simulink model "Integrated_Project"  (R2025b)
settings: Solver=ode1  StartTime=0.0  StopTime=1400  FixedStep=0.1  RelTol=1e-3
model workspace (MAT data in the model file):
  front_gain_calibration = 0.772532167539
  left_gain_calibration = 5
  right_gain_calibration = 6
values from neighbouring files (symbols this model uses):
  a_current = exp(-Ts/tau_current)    [Integrated_Project_Script.m]
  a_turn = exp(-0.1/0.5)    [Integrated_Project_Script.m]
  Charging_Current = -25    [Integrated_Project_Script.m]
  omega_TURN = double(0.5)    [Integrated_Project_Script.m]
  SOC_Critical = double(5)    [Integrated_Project_Script.m]
  SOC_Warn = double(30)    [Integrated_Project_Script.m]
  SOH_Min = double(90)    [Integrated_Project_Script.m]
  V_min = double(2.5)    [Integrated_Project_Script.m]
  vx_FORWARD = double(0.5)    [Integrated_Project_Script.m]
  vx_REDUCED = double(0.2)    [Integrated_Project_Script.m]
undefined symbols (not defined in the file or in its folder): DiscIntNeverNeededParam, dspblkCoreblockFVToolHelper, gcbh
libraries: simulink x6, sim3dlib x1, sim3dautolib x1, SignalEditorBlockLib x1
settings Model: VariantFading=off  Creator=LENOVO  LastModifiedBy=LENOVO

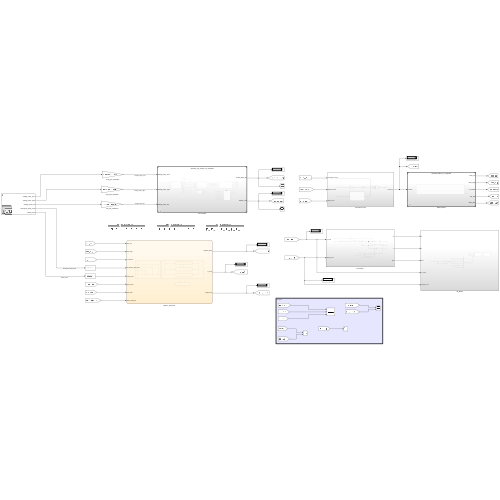
[thumbnail: Simulink's stored preview of the top-level diagram]
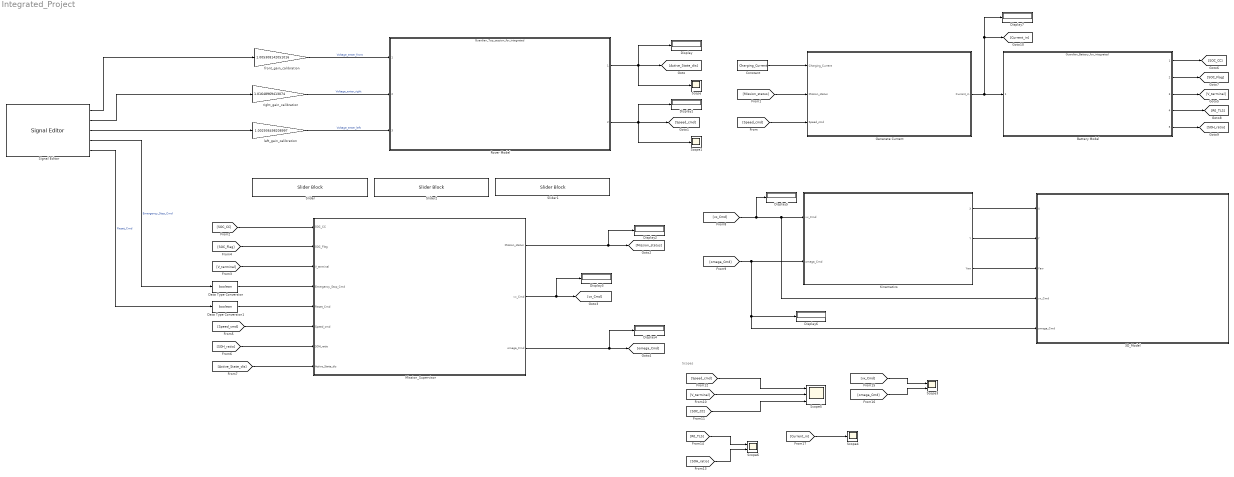
== system Integrated_Project ==
  note: Scopes
  3D_Model : Subsystem
  Battery Model : ModelReference  ModelNameDialog=Guardian_Battery_for_integrated.slx  SimulationMode=Normal  ModelReferenceVersion=1.37
  Constant : Constant  Value=Charging_Current
  Data Type Conversion : DataTypeConversion  OutDataTypeStr=boolean  SaturateOnIntegerOverflow=off  RndMeth=Floor
  Data Type Conversion1 : DataTypeConversion  OutDataTypeStr=boolean  SaturateOnIntegerOverflow=off  RndMeth=Floor
  Display{,1..7} (8 alike) : Display
  Generate Current : Subsystem
  Kinematics : Subsystem
  Mission_Supervisor : Stateflow chart  TreatAsAtomicUnit=on
  Rover Model : ModelReference  ModelNameDialog=Guardian_Top_session_for_integrated.slx  SimulationMode=Normal  ModelReferenceVersion=1.68
  Scope : Scope
  Scope1 : Scope
  Scope3 : Scope  NumInputPorts=2
      settings: ActiveDisplayYMinimum=-0.625  ActiveDisplayYMaximum=0.625  DataLoggingVariableName=ScopeData3
  Scope4 : Scope
      settings: ActiveDisplayYMinimum=-33.124999999999993  ActiveDisplayYMaximum=48.124999999999936  DataLoggingVariableName=ScopeData4
  Scope5 : Scope  NumInputPorts=3
      settings: ActiveDisplayString=3  ActiveDisplayYMinimum=45.574520890625735  ActiveDisplayYMaximum=83.82505323437492  DataLoggingVariableName=ScopeData6
  Scope6 : Scope  NumInputPorts=2
      settings: ActiveDisplayYMinimum=-1  ActiveDisplayYMaximum=1  DataLoggingVariableName=ScopeData7
  Signal Editor : SignalEditorBlockLib/Signal Editor  FileName=scenario_FINAL_ceremony.mat  ActiveScenario=ds  ActiveSignal=Voltage_enter_front  IsBus=off  OutputBusObjectStr=Bus: BusObject  SampleTime=0  ZeroCross=off  OutputAfterFinalValue=Setting to zero  Unit=inherit  PreserveSignalName=on  ApplySigPropsToAllScenarios=on  ApplySigPropsToAllSignals=off  SignalPropertySource=Dialog parameters
  Slider : SliderBlock  ScaleMax=3
  Slider1 : SliderBlock  ScaleMax=3
  Slider2 : SliderBlock  ScaleMax=3
  front_gain_calibration : Gain  Gain=1.005308142051016
  left_gain_calibration : Gain  Gain=1.002936498208997
  right_gain_calibration : Gain  Gain=1.01648969413074
  wires:
  left_gain_calibration/1 -> Rover Model/3  "Voltage_enter_left"
  front_gain_calibration/1 -> Rover Model/1  "Voltage_enter_front"
  right_gain_calibration/1 -> Rover Model/2  "Voltage_enter_right"
  Signal Editor/1 -> front_gain_calibration/1
  Signal Editor/2 -> right_gain_calibration/1
  Signal Editor/3 -> left_gain_calibration/1
  Rover Model/1 -> Display/1, Scope/1, [Active_State_dis]
  Rover Model/2 -> Scope1/1, Display1/1, [Speed_cmd]
  Signal Editor/5 -> Data Type Conversion1/1  "Reset_Cmd"
  Signal Editor/4 -> Data Type Conversion/1  "Emergency_Stop_Cmd"
  Data Type Conversion/1 -> Mission_Supervisor/4(Emergency_Stop_Cmd)
  Data Type Conversion1/1 -> Mission_Supervisor/5(Reset_Cmd)
  Mission_Supervisor/1(Mission_status) -> Display2/1, [Mission_status]
  Mission_Supervisor/2(vx_Cmd) -> Display3/1, [vx_Cmd]
  Mission_Supervisor/3(omega_Cmd) -> Display4/1, [omega_Cmd]
  [Mission_status] -> Generate Current/2(Mission_status)
  [Speed_cmd] -> Generate Current/3(Speed_cmd)
  Constant/1 -> Generate Current/1(Charging_Current)
  Generate Current/1(Current_in) -> [Current_in], Display7/1, Battery Model/1
  Battery Model/1 -> [SOC_CC]
  Battery Model/2 -> [SOC_Flag]
  Battery Model/3 -> [V_terminal]
  Battery Model/4 -> [R0_TLS]
  Battery Model/5 -> [SOH_ratio]
  [SOC_CC] -> Mission_Supervisor/1(SOC_CC)
  [V_terminal] -> Mission_Supervisor/3(V_terminal)
  [SOC_Flag] -> Mission_Supervisor/2(SOC_Flag)
  [Speed_cmd] -> Mission_Supervisor/6(Speed_cmd)
  [SOH_ratio] -> Mission_Supervisor/7(SOH_ratio)
  [Active_State_dis] -> Mission_Supervisor/8(Active_State_dis)
  [vx_Cmd] -> Display5/1, 3D_Model/4(vx_Cmd), Kinematics/1(vx_Cmd)
  [omega_Cmd] -> Display6/1, 3D_Model/5(omega_Cmd), Kinematics/2(omega_Cmd)
  Kinematics/1(X) -> 3D_Model/1(X)
  Kinematics/2(Y) -> 3D_Model/2(Y)
  Kinematics/3(Yaw) -> 3D_Model/3(Yaw)
  [Speed_cmd] -> Scope5/1
  [V_terminal] -> Scope5/2
  [SOC_CC] -> Scope5/3
  [R0_TLS] -> Scope6/1
  [SOH_ratio] -> Scope6/2
  [vx_Cmd] -> Scope3/1
  [omega_Cmd] -> Scope3/2
  [Current_in] -> Scope4/1

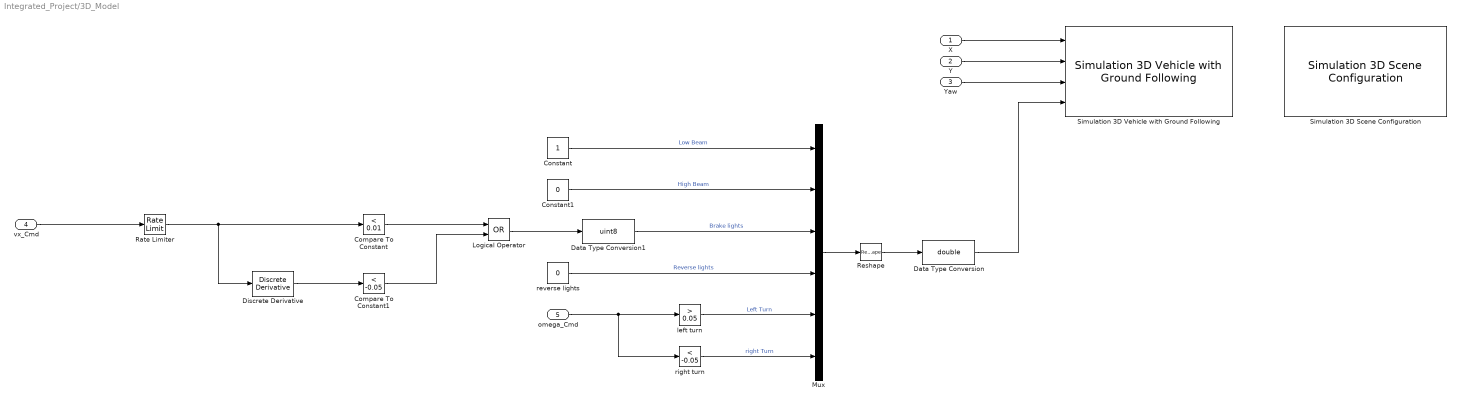
== system Integrated_Project/3D_Model ==
  X : Inport
  Y : Inport  Port=2
  Yaw : Inport  Port=3
  vx_Cmd : Inport  Port=4
  omega_Cmd : Inport  Port=5
  Compare To Constant : simulink/Logic and Bit Operations/Compare To Constant  relop=<  const=0.01  OutDataTypeStr=uint8
  Compare To Constant1 : simulink/Logic and Bit Operations/Compare To Constant  relop=<  const=-0.05  OutDataTypeStr=boolean
  Constant : Constant  OutDataTypeStr=uint8
  Constant1 : Constant  Value=0  OutDataTypeStr=uint8
  Data Type Conversion : DataTypeConversion  OutDataTypeStr=double  SaturateOnIntegerOverflow=off  RndMeth=Floor
  Data Type Conversion1 : DataTypeConversion  OutDataTypeStr=uint8  SaturateOnIntegerOverflow=off  RndMeth=Floor
  Discrete Derivative : simulink/Discrete/Discrete Derivative  gainval=1.0  ICPrevScaledInput=0.0  OutMin=[]  OutMax=[]  OutDataType=fixdt(1, 16)  OutScaling=2^-10  DoSatur=off
  Logical Operator : Logic  Operator=OR  AllPortsSameDT=off  OutDataTypeStr=boolean
  Mux : Mux  Inputs=6
  Rate Limiter : RateLimiter  RisingSlewLimit=0.5  SampleTimeMode=inherited
  Reshape : Reshape  OutputDimensions=[1 , 6]
  Simulation 3D Scene Configuration : sim3dlib/Simulation 3D Scene Configuration  Priority=0  ProjectFormat=Default Scenes  SceneDesc=Straight road  ProjectName=C:\Program Files\MATLAB\R2025b\toolbox\shared\sim3d_projects\automotive_project_windows\UE\WindowsNoEditor\VehicleSimulation.exe  ScenePath=/Game/Maps/HwStrght  EnableOpenDRIVE=off  vehTagList={'Custom';'NAGY';'Scene Origin'}  vehTag=NAGY  AttachedCameraRelativeTranslation=[0 0 0]  FreeCameraDefaultInitialTranslation=[-6, 0, 2]  AttachedCameraRelativeRotation=[0 0 0]  FreeCameraDefaultInitialRotation=[0, -15, 0]  ViewpointName=Custom  FreeCameraInitialTranslation=[0, 0, 0]  ViewpointTranslation=[0 0 0]  FreeCameraInitialRotation=[0, 0, 0]  ViewpointRotation=[0 0 0]  OpVisEn=off  Ts=0.1  EnableWindow=on  EnableRemoteAccess=off  EnableWeather=on  SunAzimuth=0.0  SunAltitude=18.0  EnableGeospatialSun=off  Latitude=0  Longitude=0  Date=2023-01-01  Time=10:30:00  GeoTimeZone=-5.0  SunDaylightSaving=off  wind=1  clouds=10  EnableVolumetricClouds=off  CloudCoverage=0  CloudAltitude=6  fog=0  rain=0  RaindropsEffect=off  SnowDensity=0  EnableGeospatial=off  TilesetSource=Earth terrain  UseTrueOrigin=off  OriginHeight=200  OriginLatitude=40.744652  OriginLongitude=-73.988864  MapStyle=Aerial  AdditionalAssetIDs=[]  UseAdvancedSunSky=off  SolarTime=11  TimeZone=-5  Day=21  Month=9  Year=2022  UseDaylightSavingTime=on  DSTStartDay=10  DSTStartMonth=3  DSTEndDay=3  DSTEndMonth=11  DSTSwitchHour=2  sensorTag=MainCamera1  sensorId=1  sensorName=MainCamera1  mountLoc=Origin  offsetFlag=off  tmountOffset=[0, 0, 0]  rmountOffset=[0, 0, 0]  HorizontalResolution=1280  VerticalResolution=720  HorizontalFOV=60  mountPoint=[0 0 0]  mountOrientation=[0 0 0]  aMode=5  ID=1  GeoTrigger=Inactive  ViewNameList={'Custom'}  ViewTranslationList={'[0 0 0]'}  ViewRotationList={'[0 0 0]'}
      settings: LibrarySourceBlock=sl3dlib/Simulation 3D/Environment/Simulation 3D Scene Configuration
  Simulation 3D Vehicle with Ground Following : sim3dautolib/Simulation 3D Vehicle with Ground Following  Priority=-1  PassVehMesh=Muscle car  MeshPath=/MathWorksAutomotiveContent/Vehicles/Muscle/Meshes/SK_MuscleCar.SK_MuscleCar  TrackWidth=1.9  WheelBase=3  WheelRadius=0.35  VehColor=Black  CoordinateSystem=ISO8855  InitialPos=[0, 0, 0]  InitialRot=[0, 0, 0]  ActorName=NAGY  SampleTime=0.1  ActorType=SimulinkVehicle  ID=C  aMode=3  ActorTag=NAGY  CoordinateScheme=0  VehLightsControl=on  HeadlightColor=[ 1, 0.95 , 0.7 ]  HighBeamIntensity=60000  LowBeamIntensity=20000  HighBeamConeAngle=35  LowBeamConeAngle=35  LeftHeadlightOrientation=[ -5, 0 ]  RightHeadlightOrientation=[ -5, 0 ]  BrakelightIntensity=1500  ReverselightIntensity=1500  SignallightIntensity=5000  SignallightPeriod=0.8  SignalPulseWidth=50  TransformOutportEnabled=off
      settings: LibrarySourceBlock=drivingsim3d/Simulation 3D Vehicle with Ground Following
  left turn : simulink/Logic and Bit Operations/Compare To Constant  relop=>  const=0.05  OutDataTypeStr=uint8
  reverse lights : Constant  Value=0  OutDataTypeStr=uint8
  right turn : simulink/Logic and Bit Operations/Compare To Constant  relop=<  const=-0.05  OutDataTypeStr=uint8
  wires:
  Yaw/1 -> Simulation 3D Vehicle with Ground Following/3
  Y/1 -> Simulation 3D Vehicle with Ground Following/2
  X/1 -> Simulation 3D Vehicle with Ground Following/1
  Data Type Conversion/1 -> Simulation 3D Vehicle with Ground Following/4
  Constant1/1 -> Mux/2  "High Beam"
  right turn/1 -> Mux/6  "right Turn"
  reverse lights/1 -> Mux/4  "Reverse lights"
  omega_Cmd/1 -> right turn/1, left turn/1
  Constant/1 -> Mux/1  "Low Beam"
  Compare To Constant/1 -> Logical Operator/1
  Mux/1 -> Reshape/1
  vx_Cmd/1 -> Rate Limiter/1
  left turn/1 -> Mux/5  "Left Turn"
  Reshape/1 -> Data Type Conversion/1
  Rate Limiter/1 -> Discrete Derivative/1, Compare To Constant/1
  Logical Operator/1 -> Data Type Conversion1/1
  Discrete Derivative/1 -> Compare To Constant1/1
  Compare To Constant1/1 -> Logical Operator/2
  Data Type Conversion1/1 -> Mux/3  "Brake lights"

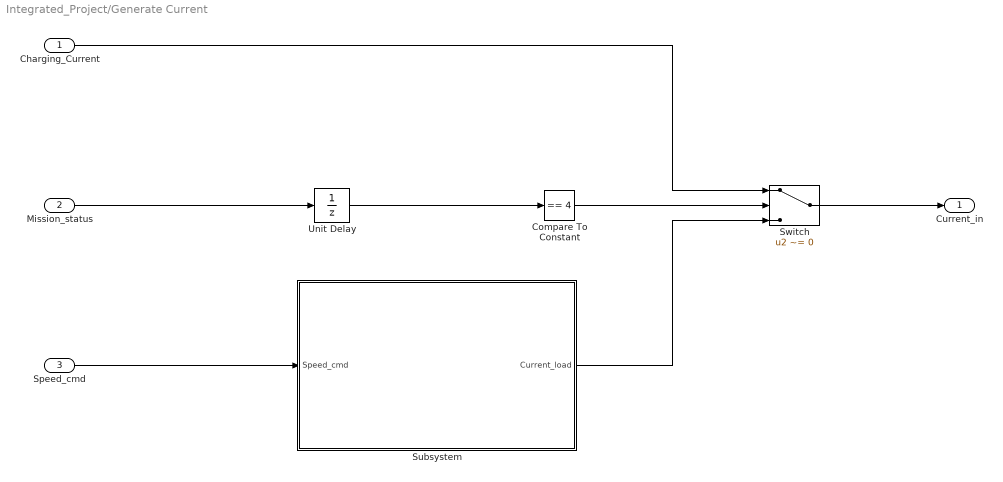
== system Integrated_Project/Generate Current ==
  Charging_Current : Inport
  Mission_status : Inport  Port=2
  Speed_cmd : Inport  Port=3
  Compare To Constant : simulink/Logic and Bit Operations/Compare To Constant  relop===  const=4  OutDataTypeStr=boolean
  Subsystem : Subsystem
  Switch : Switch  Criteria=u2 ~= 0  Threshold=4  SaturateOnIntegerOverflow=off  InputSameDT=off
  Unit Delay : UnitDelay  SampleTime=-1  HasFrameUpgradeWarning=on
  Current_in : Outport
  wires:
  Mission_status/1 -> Unit Delay/1
  Unit Delay/1 -> Compare To Constant/1
  Compare To Constant/1 -> Switch/2
  Charging_Current/1 -> Switch/1
  Speed_cmd/1 -> Subsystem/1(Speed_cmd)
  Subsystem/1(Current_load) -> Switch/3
  Switch/1 -> Current_in/1

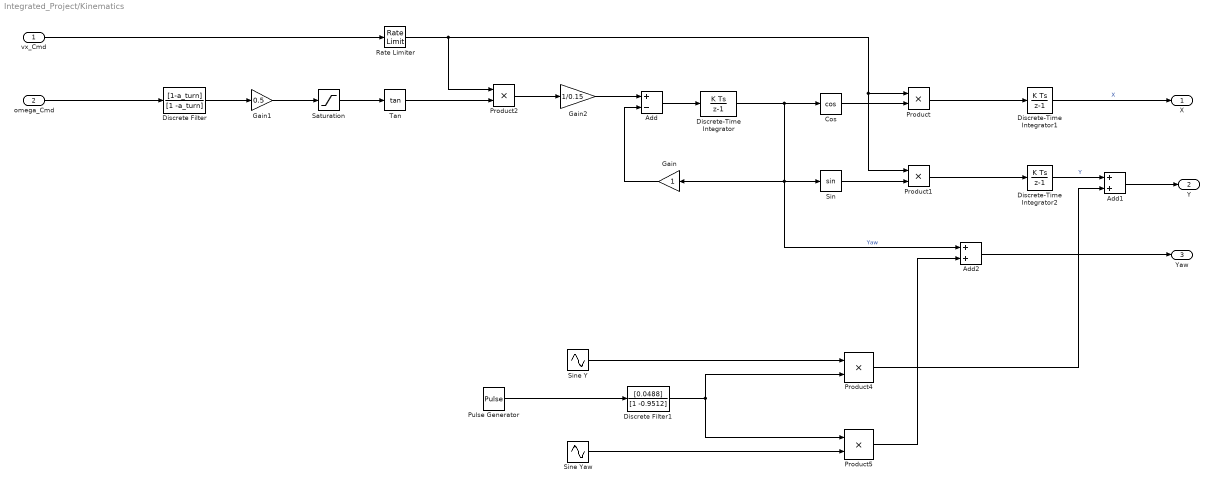
== system Integrated_Project/Kinematics ==
  vx_Cmd : Inport
  omega_Cmd : Inport  Port=2
  Add : Sum  Inputs=+-
  Add1 : Sum
  Add2 : Sum
  Cos : Trigonometry  Operator=cos
  Discrete Filter : DiscreteFilter  LoadFcn=dspblkCoreblockFVToolHelper(gcbh,'load');  Numerator=[1-a_turn]  Denominator=[1 -a_turn]
      settings: CopyFcn=dspblkCoreblockFVToolHelper(gcbh,'copy');  DeleteFcn=dspblkCoreblockFVToolHelper(gcbh,'close');  ModelCloseFcn=dspblkCoreblockFVToolHelper(gcbh,'close');  PreSaveFcn=dspblkCoreblockFVToolHelper(gcbh,'presave');  PostSaveFcn=dspblkCoreblockFVToolHelper(gcbh,'postsave');  CloseFcn=dspblkCoreblockFVToolHelper(gcbh,'close');
  Discrete Filter1 : DiscreteFilter  LoadFcn=dspblkCoreblockFVToolHelper(gcbh,'load');  Numerator=[0.0488]  Denominator=[1 -0.9512]
      settings: CopyFcn=dspblkCoreblockFVToolHelper(gcbh,'copy');  DeleteFcn=dspblkCoreblockFVToolHelper(gcbh,'close');  ModelCloseFcn=dspblkCoreblockFVToolHelper(gcbh,'close');  PreSaveFcn=dspblkCoreblockFVToolHelper(gcbh,'presave');  PostSaveFcn=dspblkCoreblockFVToolHelper(gcbh,'postsave');  CloseFcn=dspblkCoreblockFVToolHelper(gcbh,'close');
  Discrete-Time Integrator : DiscreteIntegrator  SampleTime=-1  LimitOutput=on  UpperSaturationLimit=0.4  LowerSaturationLimit=-0.4  ICPrevOutput=DiscIntNeverNeededParam  ICPrevScaledInput=DiscIntNeverNeededParam
  Discrete-Time Integrator1 : DiscreteIntegrator  SampleTime=-1  ICPrevOutput=DiscIntNeverNeededParam  ICPrevScaledInput=DiscIntNeverNeededParam
  Discrete-Time Integrator2 : DiscreteIntegrator  SampleTime=-1  ICPrevOutput=DiscIntNeverNeededParam  ICPrevScaledInput=DiscIntNeverNeededParam
  Gain : Gain
  Gain1 : Gain  Gain=0.5
  Gain2 : Gain  Gain=1/0.15
  Product{,1..2,4..5} (5 alike) : Product
  Pulse Generator : DiscretePulseGenerator  PulseType=Time based  Period=1000  PulseWidth=2.4  PhaseDelay=30
  Rate Limiter : RateLimiter  RisingSlewLimit=0.5  SampleTimeMode=inherited
  Saturation : Saturate
  Sin : Trigonometry
  Sine Y : Sin  Amplitude=0.6  Frequency=0.6  SampleTime=0.1
  Sine Yaw : Sin  Amplitude=0.5  Frequency=0.6  Phase=pi/2  SampleTime=0.1
  Tan : Trigonometry  Operator=tan
  X : Outport
  Y : Outport  Port=2
  Yaw : Outport  Port=3
  wires:
  vx_Cmd/1 -> Rate Limiter/1
  omega_Cmd/1 -> Discrete Filter/1
  Discrete-Time Integrator/1 -> Add2/1, Gain/1, Sin/1, Cos/1  "Yaw"
  Cos/1 -> Product/2
  Product/1 -> Discrete-Time Integrator1/1
  Discrete-Time Integrator1/1 -> X/1  "X"
  Sin/1 -> Product1/2
  Product1/1 -> Discrete-Time Integrator2/1
  Discrete-Time Integrator2/1 -> Add1/1  "Y"
  Gain/1 -> Add/2
  Add/1 -> Discrete-Time Integrator/1
  Rate Limiter/1 -> Product2/1, Product1/1, Product/1
  Discrete Filter/1 -> Gain1/1
  Gain1/1 -> Saturation/1
  Saturation/1 -> Tan/1
  Tan/1 -> Product2/2
  Product2/1 -> Gain2/1
  Gain2/1 -> Add/1
  Pulse Generator/1 -> Discrete Filter1/1
  Sine Y/1 -> Product4/1
  Sine Yaw/1 -> Product5/2
  Add1/1 -> Y/1
  Add2/1 -> Yaw/1
  Discrete Filter1/1 -> Product4/2, Product5/1
  Product4/1 -> Add1/2
  Product5/1 -> Add2/2

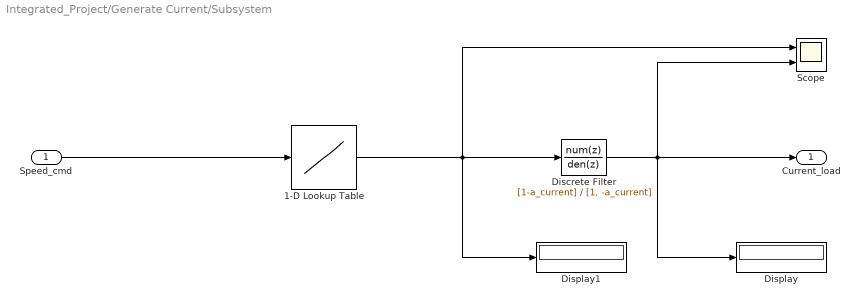
== system Integrated_Project/Generate Current/Subsystem ==
  Speed_cmd : Inport
  1-D Lookup Table : Lookup_n-D  NumberOfTableDimensions=1  BreakpointsForDimension1=[0 , 25 , 50 , 100]  Table=[0, 10, 20, 40]  InternalRulePriority=Speed  RndMeth=Simplest
  Discrete Filter : DiscreteFilter  LoadFcn=dspblkCoreblockFVToolHelper(gcbh,'load');  Numerator=[1-a_current]  Denominator=[1, -a_current]
      settings: CopyFcn=dspblkCoreblockFVToolHelper(gcbh,'copy');  DeleteFcn=dspblkCoreblockFVToolHelper(gcbh,'close');  ModelCloseFcn=dspblkCoreblockFVToolHelper(gcbh,'close');  PreSaveFcn=dspblkCoreblockFVToolHelper(gcbh,'presave');  PostSaveFcn=dspblkCoreblockFVToolHelper(gcbh,'postsave');  CloseFcn=dspblkCoreblockFVToolHelper(gcbh,'close');
  Display : Display
  Display1 : Display
  Scope : Scope  NumInputPorts=2
      settings: DataLoggingVariableName=ScopeData5
  Current_load : Outport
  wires:
  Speed_cmd/1 -> 1-D Lookup Table/1
  1-D Lookup Table/1 -> Display1/1, Scope/1, Discrete Filter/1
  Discrete Filter/1 -> Display/1, Scope/2, Current_load/1

== stateflow chart Integrated_Project/Mission_Supervisor ==
  state [vx , omega] = StateToKinematics (state , vx_scale , omega_scale) [function]
    (default) -> (junction 71) : % kinematics
    (junction 71) -> (junction 72) [order 1] : [state == 1]
    (junction 71) -> (junction 73) [order 2]
    (junction 72) -> (junction 80) : {vx = vx_scale * (Speed_cmd/100); omega=0;}
    (junction 73) -> (junction 74) [order 1] : [state == 2]
    (junction 73) -> (junction 75) [order 2]
    (junction 74) -> (junction 79) : {vx = 0; omega = omega_scale;}
    (junction 75) -> (junction 76) [order 1] : [state == 3]
    (junction 75) -> (junction 77) [order 2] : {vx = 0; omega = 0;}
    (junction 76) -> (junction 78) : {vx = 0; omega = -omega_scale;}
    (junction 78) -> (junction 77)
    (junction 79) -> (junction 78)
    (junction 80) -> (junction 79)
    (junction 77) -> (junction 81)
  state operating
    (history)
    state NOMINAL
      entry:
      Mission_status = 1;
      du:
      [vx_Cmd , omega_Cmd] = StateToKinematics (Active_State_dis , vx_FORWARD ,  omega_TURN)
    state LOW_POWER
      entry:
      Mission_status = 2;
      du:
      [vx_Cmd , omega_Cmd] = StateToKinematics (Active_State_dis , vx_REDUCED ,  omega_TURN)
    state CELL_FAULT
      entry:
      Mission_status = 3;
      du:
      [vx_Cmd , omega_Cmd] = StateToKinematics (Active_State_dis , vx_REDUCED ,  omega_TURN)
    (default) -> NOMINAL
    NOMINAL -> (junction 17) [order 1] : [SOC_Flag == true]
    (junction 32) -> NOMINAL
    (junction 17) -> (junction 19)
    (junction 29) -> (junction 32) [order 2] : [SOC_CC >= SOC_Warn && SOH_ratio >= SOH_Min]
    NOMINAL -> LOW_POWER [order 2] : [SOC_CC >= SOC_Warn && SOH_ratio >= SOH_Min]
    LOW_POWER -> NOMINAL : [SOC_CC < SOC_Warn || SOH_ratio < SOH_Min]
    (junction 29) -> LOW_POWER [order 1] : [SOC_CC < SOC_Warn || SOH_ratio < SOH_Min]
    (junction 27) -> (junction 29)
    (junction 19) -> LOW_POWER [order 1] : [SOC_Flag == true]
    (junction 19) -> (junction 22) [order 2]
    CELL_FAULT -> (junction 27) : [SOC_Flag == false]
    (junction 22) -> CELL_FAULT
  state RTB_STOP
    entry:
    Mission_status = 4;
    vx_Cmd = 0;
    omega_Cmd = 0;
  (default) -> operating
  operating -> RTB_STOP : [Emergency_Stop_Cmd == true ||SOC_CC < SOC_Critical || V_terminal < V_min]
  RTB_STOP -> operating : [Reset_Cmd == true]
  data: state function_input; vx_scale function_input; omega_scale function_input; vx function_output; omega function_output; SOC_CC input double; SOC_Flag input boolean; V_terminal input double; Emergency_Stop_Cmd input boolean; Reset_Cmd input boolean; Mission_status output int32; vx_Cmd output double; omega_Cmd output double; Speed_cmd input double; SOH_ratio input double; SOH_Min parameter double; SOC_Critical parameter double; SOC_Warn parameter double; V_min parameter double; Active_State_dis input int32; omega_TURN parameter double; vx_FORWARD parameter double; vx_REDUCED parameter double
